simulink model "adc_16g_asnt"  (R2018a)
settings: Solver=VariableStepAuto  StartTime=0.0  StopTime=10.0  RelTol=1e-3
libraries: xbsIndex_r4 x65
settings Model: Creator=jkocz  LastModifiedBy=wei
settings CodeAppCC: StateflowObjectComments=on

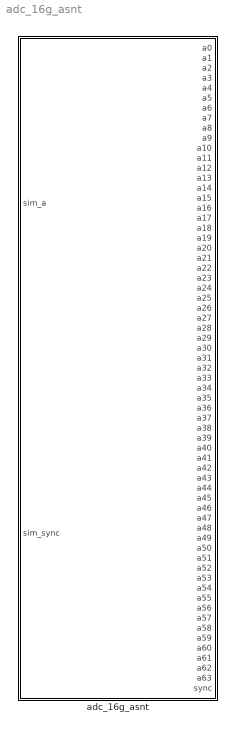
== system adc_16g_asnt ==
  adc_16g_asnt : Subsystem  Tag=xps:adc_4x16g_asnt  AncestorBlock=xps_adc/ADCs/adc_5g_e2v  mask(asnt_16g_adc){channel_sel=0}
      mask prompts: channel_sel "Channel Selection"
      mask init:
      | adc_16g_asnt_init(gcb);
      mask TypeOptions channel_sel: 0 | 1 | 2 | 3

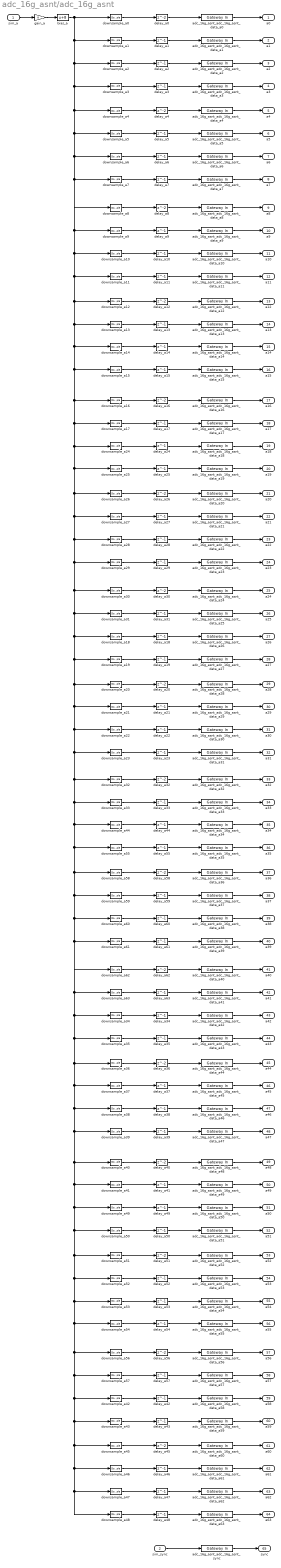
== system adc_16g_asnt/adc_16g_asnt ==
  sim_a : Inport
  sim_sync : Inport  Port=2
  adc_16g_asnt_adc_16g_asnt_data_a{0..63} (64 alike) : xbsIndex_r4/Gateway In  gui_display_data_type=Fixed-point  arith_type=Unsigned  n_bits=4  bin_pt=0  preci_type=Single  exp_width=8  frac_width=24  rows=1  columns=1  quantization=Truncate  overflow=Wrap  period=1  UseAsADC=off  ADCChannel='1'  interface=None  automatic_assignment=on  address_offset=hex2dec('00')  intf_name=''  intf_description=''  default_value=0  timing_constraint=None  locs_specified=off  LOCs={}  io_standard={}  inherit_from_input=off  hdl_port=on  dbl_ovrd=off  block_type=gatewayin
  adc_16g_asnt_adc_16g_asnt_sync : xbsIndex_r4/Gateway In  gui_display_data_type=Fixed-point  arith_type=Boolean  n_bits=16  bin_pt=14  preci_type=Single  exp_width=8  frac_width=24  rows=1  columns=1  quantization="Round  (unbiased: +/- Inf)"  overflow=Saturate  period=1  UseAsADC=off  ADCChannel='1'  interface=None  automatic_assignment=on  address_offset=hex2dec('00')  intf_name=''  intf_description=''  default_value=0  timing_constraint=None  locs_specified=off  LOCs={}  io_standard={}  inherit_from_input=off  hdl_port=on  dbl_ovrd=off  block_type=gatewayin
  bias_a : Bias  Bias=8  SaturateOnIntegerOverflow=on
  delay_a{0,4,8,12,16,20,26,30,32,36,40,45,51,56,58,62} (16 alike) : Delay  InitialCondition=0  InputProcessing=Inherited
  delay_a{1..3,5..7,9..11,13..15,17..19,21..25,27..29,31,33..35,37..39,41..44,46..50,52..55,57,59..61,63} (48 alike) : Delay  DelayLength=1  InitialCondition=0  InputProcessing=Inherited
  downsample_a{0,4,8,12,16,20,26,30,32,36,40,45,51,56,58,62} (16 alike) : DownSample  N=64  RateOptions=Allow multirate processing
  downsample_a{1,5,9,13,17,21,27,31,33,37,41,46,52,57,59,63} (16 alike) : DownSample  N=64  phase=1  RateOptions=Allow multirate processing
  downsample_a{2,6,10,14,18,22,24,28,34,38,42,44,47,49,53,60} (16 alike) : DownSample  N=64  phase=2  RateOptions=Allow multirate processing
  downsample_a{3,7,11,15,19,23,25,29,35,39,43,48,50,54..55,61} (16 alike) : DownSample  N=64  phase=3  RateOptions=Allow multirate processing
  gain_a : Gain  Gain=8  SaturateOnIntegerOverflow=on  OutDataTypeStr=Inherit: Same as input  ParamDataTypeStr=Inherit: Same as input
  a0 : Outport
  a1 : Outport  Port=2
  a2 : Outport  Port=3
  a3 : Outport  Port=4
  a4 : Outport  Port=5
  a5 : Outport  Port=6
  a6 : Outport  Port=7
  a7 : Outport  Port=8
  a8 : Outport  Port=9
  a9 : Outport  Port=10
  a10 : Outport  Port=11
  a11 : Outport  Port=12
  a12 : Outport  Port=13
  a13 : Outport  Port=14
  a14 : Outport  Port=15
  a15 : Outport  Port=16
  a16 : Outport  Port=17
  a17 : Outport  Port=18
  a18 : Outport  Port=19
  a19 : Outport  Port=20
  a20 : Outport  Port=21
  a21 : Outport  Port=22
  a22 : Outport  Port=23
  a23 : Outport  Port=24
  a24 : Outport  Port=25
  a25 : Outport  Port=26
  a26 : Outport  Port=27
  a27 : Outport  Port=28
  a28 : Outport  Port=29
  a29 : Outport  Port=30
  a30 : Outport  Port=31
  a31 : Outport  Port=32
  a32 : Outport  Port=33
  a33 : Outport  Port=34
  a34 : Outport  Port=35
  a35 : Outport  Port=36
  a36 : Outport  Port=37
  a37 : Outport  Port=38
  a38 : Outport  Port=39
  a39 : Outport  Port=40
  a40 : Outport  Port=41
  a41 : Outport  Port=42
  a42 : Outport  Port=43
  a43 : Outport  Port=44
  a44 : Outport  Port=45
  a45 : Outport  Port=46
  a46 : Outport  Port=47
  a47 : Outport  Port=48
  a48 : Outport  Port=49
  a49 : Outport  Port=50
  a50 : Outport  Port=51
  a51 : Outport  Port=52
  a52 : Outport  Port=53
  a53 : Outport  Port=54
  a54 : Outport  Port=55
  a55 : Outport  Port=56
  a56 : Outport  Port=57
  a57 : Outport  Port=58
  a58 : Outport  Port=59
  a59 : Outport  Port=60
  a60 : Outport  Port=61
  a61 : Outport  Port=62
  a62 : Outport  Port=63
  a63 : Outport  Port=64
  sync : Outport  Port=65
  wires:
  sim_sync/1 -> adc_16g_asnt_adc_16g_asnt_sync/1
  adc_16g_asnt_adc_16g_asnt_data_a3/1 -> a3/1
  delay_a3/1 -> adc_16g_asnt_adc_16g_asnt_data_a3/1
  downsample_a3/1 -> delay_a3/1
  adc_16g_asnt_adc_16g_asnt_data_a2/1 -> a2/1
  delay_a2/1 -> adc_16g_asnt_adc_16g_asnt_data_a2/1
  downsample_a2/1 -> delay_a2/1
  adc_16g_asnt_adc_16g_asnt_data_a1/1 -> a1/1
  delay_a1/1 -> adc_16g_asnt_adc_16g_asnt_data_a1/1
  downsample_a1/1 -> delay_a1/1
  adc_16g_asnt_adc_16g_asnt_data_a0/1 -> a0/1
  delay_a0/1 -> adc_16g_asnt_adc_16g_asnt_data_a0/1
  downsample_a0/1 -> delay_a0/1
  gain_a/1 -> bias_a/1
  sim_a/1 -> gain_a/1
  adc_16g_asnt_adc_16g_asnt_data_a6/1 -> a6/1
  delay_a4/1 -> adc_16g_asnt_adc_16g_asnt_data_a4/1
  adc_16g_asnt_adc_16g_asnt_data_a7/1 -> a7/1
  downsample_a5/1 -> delay_a5/1
  adc_16g_asnt_adc_16g_asnt_data_a4/1 -> a4/1
  downsample_a7/1 -> delay_a7/1
  adc_16g_asnt_adc_16g_asnt_data_a5/1 -> a5/1
  downsample_a6/1 -> delay_a6/1
  delay_a5/1 -> adc_16g_asnt_adc_16g_asnt_data_a5/1
  delay_a7/1 -> adc_16g_asnt_adc_16g_asnt_data_a7/1
  delay_a6/1 -> adc_16g_asnt_adc_16g_asnt_data_a6/1
  downsample_a4/1 -> delay_a4/1
  adc_16g_asnt_adc_16g_asnt_data_a10/1 -> a10/1
  delay_a8/1 -> adc_16g_asnt_adc_16g_asnt_data_a8/1
  adc_16g_asnt_adc_16g_asnt_data_a11/1 -> a11/1
  downsample_a9/1 -> delay_a9/1
  adc_16g_asnt_adc_16g_asnt_data_a8/1 -> a8/1
  downsample_a11/1 -> delay_a11/1
  adc_16g_asnt_adc_16g_asnt_data_a9/1 -> a9/1
  downsample_a10/1 -> delay_a10/1
  delay_a9/1 -> adc_16g_asnt_adc_16g_asnt_data_a9/1
  delay_a11/1 -> adc_16g_asnt_adc_16g_asnt_data_a11/1
  delay_a10/1 -> adc_16g_asnt_adc_16g_asnt_data_a10/1
  downsample_a8/1 -> delay_a8/1
  adc_16g_asnt_adc_16g_asnt_data_a14/1 -> a14/1
  delay_a12/1 -> adc_16g_asnt_adc_16g_asnt_data_a12/1
  adc_16g_asnt_adc_16g_asnt_data_a15/1 -> a15/1
  downsample_a13/1 -> delay_a13/1
  adc_16g_asnt_adc_16g_asnt_data_a12/1 -> a12/1
  downsample_a15/1 -> delay_a15/1
  adc_16g_asnt_adc_16g_asnt_data_a13/1 -> a13/1
  downsample_a14/1 -> delay_a14/1
  delay_a13/1 -> adc_16g_asnt_adc_16g_asnt_data_a13/1
  delay_a15/1 -> adc_16g_asnt_adc_16g_asnt_data_a15/1
  delay_a14/1 -> adc_16g_asnt_adc_16g_asnt_data_a14/1
  downsample_a12/1 -> delay_a12/1
  delay_a25/1 -> adc_16g_asnt_adc_16g_asnt_data_a19/1
  delay_a31/1 -> adc_16g_asnt_adc_16g_asnt_data_a25/1
  adc_16g_asnt_adc_16g_asnt_data_a27/1 -> a27/1
  adc_16g_asnt_adc_16g_asnt_data_a21/1 -> a21/1
  downsample_a29/1 -> delay_a29/1
  downsample_a27/1 -> delay_a27/1
  adc_16g_asnt_adc_16g_asnt_data_a20/1 -> a20/1
  adc_16g_asnt_adc_16g_asnt_data_a31/1 -> a31/1
  delay_a18/1 -> adc_16g_asnt_adc_16g_asnt_data_a26/1
  downsample_a21/1 -> delay_a21/1
  adc_16g_asnt_adc_16g_asnt_data_a25/1 -> a25/1
  adc_16g_asnt_adc_16g_asnt_data_a22/1 -> a22/1
  adc_16g_asnt_adc_16g_asnt_data_a18/1 -> a18/1
  downsample_a19/1 -> delay_a19/1
  delay_a23/1 -> adc_16g_asnt_adc_16g_asnt_data_a31/1
  downsample_a22/1 -> delay_a22/1
  downsample_a26/1 -> delay_a26/1
  delay_a28/1 -> adc_16g_asnt_adc_16g_asnt_data_a22/1
  delay_a21/1 -> adc_16g_asnt_adc_16g_asnt_data_a29/1
  delay_a30/1 -> adc_16g_asnt_adc_16g_asnt_data_a24/1
  downsample_a18/1 -> delay_a18/1
  downsample_a30/1 -> delay_a30/1
  downsample_a28/1 -> delay_a28/1
  downsample_a31/1 -> delay_a31/1
  delay_a27/1 -> adc_16g_asnt_adc_16g_asnt_data_a21/1
  delay_a22/1 -> adc_16g_asnt_adc_16g_asnt_data_a30/1
  adc_16g_asnt_adc_16g_asnt_data_a24/1 -> a24/1
  delay_a20/1 -> adc_16g_asnt_adc_16g_asnt_data_a28/1
  downsample_a20/1 -> delay_a20/1
  downsample_a23/1 -> delay_a23/1
  adc_16g_asnt_adc_16g_asnt_data_a26/1 -> a26/1
  adc_16g_asnt_adc_16g_asnt_data_a29/1 -> a29/1
  delay_a19/1 -> adc_16g_asnt_adc_16g_asnt_data_a27/1
  delay_a29/1 -> adc_16g_asnt_adc_16g_asnt_data_a23/1
  adc_16g_asnt_adc_16g_asnt_data_a23/1 -> a23/1
  downsample_a25/1 -> delay_a25/1
  downsample_a24/1 -> delay_a24/1
  adc_16g_asnt_adc_16g_asnt_data_a17/1 -> a17/1
  delay_a17/1 -> adc_16g_asnt_adc_16g_asnt_data_a17/1
  adc_16g_asnt_adc_16g_asnt_data_a16/1 -> a16/1
  downsample_a17/1 -> delay_a17/1
  adc_16g_asnt_adc_16g_asnt_data_a19/1 -> a19/1
  delay_a16/1 -> adc_16g_asnt_adc_16g_asnt_data_a16/1
  delay_a24/1 -> adc_16g_asnt_adc_16g_asnt_data_a18/1
  downsample_a16/1 -> delay_a16/1
  adc_16g_asnt_adc_16g_asnt_data_a28/1 -> a28/1
  adc_16g_asnt_adc_16g_asnt_data_a30/1 -> a30/1
  delay_a26/1 -> adc_16g_asnt_adc_16g_asnt_data_a20/1
  downsample_a59/1 -> delay_a59/1
  delay_a42/1 -> adc_16g_asnt_adc_16g_asnt_data_a58/1
  adc_16g_asnt_adc_16g_asnt_data_a36/1 -> a36/1
  adc_16g_asnt_adc_16g_asnt_data_a38/1 -> a38/1
  adc_16g_asnt_adc_16g_asnt_data_a42/1 -> a42/1
  downsample_a61/1 -> delay_a61/1
  downsample_a46/1 -> delay_a46/1
  delay_a53/1 -> adc_16g_asnt_adc_16g_asnt_data_a54/1
  downsample_a37/1 -> delay_a37/1
  delay_a39/1 -> adc_16g_asnt_adc_16g_asnt_data_a47/1
  downsample_a49/1 -> delay_a49/1
  adc_16g_asnt_adc_16g_asnt_data_a56/1 -> a56/1
  downsample_a50/1 -> delay_a50/1
  delay_a37/1 -> adc_16g_asnt_adc_16g_asnt_data_a45/1
  adc_16g_asnt_adc_16g_asnt_data_a47/1 -> a47/1
  delay_a34/1 -> adc_16g_asnt_adc_16g_asnt_data_a42/1
  downsample_a63/1 -> delay_a63/1
  delay_a50/1 -> adc_16g_asnt_adc_16g_asnt_data_a51/1
  downsample_a43/1 -> delay_a43/1
  downsample_a42/1 -> delay_a42/1
  delay_a38/1 -> adc_16g_asnt_adc_16g_asnt_data_a46/1
  downsample_a45/1 -> delay_a45/1
  downsample_a52/1 -> delay_a52/1
  downsample_a58/1 -> delay_a58/1
  downsample_a35/1 -> delay_a35/1
  adc_16g_asnt_adc_16g_asnt_data_a62/1 -> a62/1
  downsample_a56/1 -> delay_a56/1
  downsample_a54/1 -> delay_a54/1
  delay_a62/1 -> adc_16g_asnt_adc_16g_asnt_data_a40/1
  delay_a61/1 -> adc_16g_asnt_adc_16g_asnt_data_a39/1
  adc_16g_asnt_adc_16g_asnt_data_a60/1 -> a60/1
  adc_16g_asnt_adc_16g_asnt_data_a37/1 -> a37/1
  delay_a56/1 -> adc_16g_asnt_adc_16g_asnt_data_a56/1
  downsample_a60/1 -> delay_a60/1
  delay_a63/1 -> adc_16g_asnt_adc_16g_asnt_data_a41/1
  delay_a47/1 -> adc_16g_asnt_adc_16g_asnt_data_a62/1
  adc_16g_asnt_adc_16g_asnt_data_a43/1 -> a43/1
  downsample_a51/1 -> delay_a51/1
  downsample_a40/1 -> delay_a40/1
  adc_16g_asnt_adc_16g_asnt_data_a40/1 -> a40/1
  adc_16g_asnt_adc_16g_asnt_data_a61/1 -> a61/1
  adc_16g_asnt_adc_16g_asnt_data_a53/1 -> a53/1
  adc_16g_asnt_adc_16g_asnt_data_a63/1 -> a63/1
  adc_16g_asnt_adc_16g_asnt_data_a55/1 -> a55/1
  downsample_a62/1 -> delay_a62/1
  delay_a41/1 -> adc_16g_asnt_adc_16g_asnt_data_a49/1
  adc_16g_asnt_adc_16g_asnt_data_a39/1 -> a39/1
  adc_16g_asnt_adc_16g_asnt_data_a52/1 -> a52/1
  delay_a60/1 -> adc_16g_asnt_adc_16g_asnt_data_a38/1
  delay_a46/1 -> adc_16g_asnt_adc_16g_asnt_data_a61/1
  delay_a59/1 -> adc_16g_asnt_adc_16g_asnt_data_a37/1
  adc_16g_asnt_adc_16g_asnt_data_a58/1 -> a58/1
  adc_16g_asnt_adc_16g_asnt_data_a48/1 -> a48/1
  delay_a45/1 -> adc_16g_asnt_adc_16g_asnt_data_a60/1
  delay_a35/1 -> adc_16g_asnt_adc_16g_asnt_data_a43/1
  delay_a36/1 -> adc_16g_asnt_adc_16g_asnt_data_a44/1
  adc_16g_asnt_adc_16g_asnt_data_a57/1 -> a57/1
  downsample_a39/1 -> delay_a39/1
  downsample_a32/1 -> delay_a32/1
  downsample_a34/1 -> delay_a34/1
  downsample_a38/1 -> delay_a38/1
  adc_16g_asnt_adc_16g_asnt_data_a44/1 -> a44/1
  downsample_a36/1 -> delay_a36/1
  adc_16g_asnt_adc_16g_asnt_data_a59/1 -> a59/1
  delay_a40/1 -> adc_16g_asnt_adc_16g_asnt_data_a48/1
  delay_a48/1 -> adc_16g_asnt_adc_16g_asnt_data_a63/1
  adc_16g_asnt_adc_16g_asnt_data_a41/1 -> a41/1
  adc_16g_asnt_adc_16g_asnt_data_a45/1 -> a45/1
  downsample_a41/1 -> delay_a41/1
  adc_16g_asnt_adc_16g_asnt_data_a50/1 -> a50/1
  downsample_a47/1 -> delay_a47/1
  delay_a32/1 -> adc_16g_asnt_adc_16g_asnt_data_a32/1
  adc_16g_asnt_adc_16g_asnt_data_a51/1 -> a51/1
  adc_16g_asnt_adc_16g_asnt_data_a49/1 -> a49/1
  downsample_a53/1 -> delay_a53/1
  delay_a52/1 -> adc_16g_asnt_adc_16g_asnt_data_a53/1
  downsample_a57/1 -> delay_a57/1
  adc_16g_asnt_adc_16g_asnt_data_a54/1 -> a54/1
  delay_a43/1 -> adc_16g_asnt_adc_16g_asnt_data_a59/1
  delay_a49/1 -> adc_16g_asnt_adc_16g_asnt_data_a50/1
  delay_a57/1 -> adc_16g_asnt_adc_16g_asnt_data_a57/1
  delay_a51/1 -> adc_16g_asnt_adc_16g_asnt_data_a52/1
  downsample_a55/1 -> delay_a55/1
  downsample_a44/1 -> delay_a44/1
  adc_16g_asnt_adc_16g_asnt_data_a33/1 -> a33/1
  delay_a33/1 -> adc_16g_asnt_adc_16g_asnt_data_a33/1
  adc_16g_asnt_adc_16g_asnt_data_a32/1 -> a32/1
  downsample_a33/1 -> delay_a33/1
  adc_16g_asnt_adc_16g_asnt_data_a35/1 -> a35/1
  bias_a/1 -> downsample_a44/1, downsample_a46/1, downsample_a47/1, downsample_a48/1, downsample_a45/1, downsample_a43/1, downsample_a42/1, downsample_a57/1, downsample_a56/1, downsample_a54/1, downsample_a53/1, downsample_a52/1, downsample_a51/1, downsample_a50/1, downsample_a49/1, downsample_a41/1, downsample_a40/1, downsample_a39/1, downsample_a38/1, downsample_a37/1, downsample_a36/1, downsample_a35/1, downsample_a34/1, downsample_a63/1, downsample_a32/1, downsample_a33/1, downsample_a55/1, downsample_a58/1, downsample_a59/1, downsample_a60/1, downsample_a62/1, downsample_a61/1, downsample_a23/1, downsample_a22/1, downsample_a21/1, downsample_a20/1, downsample_a19/1, downsample_a18/1, downsample_a31/1, downsample_a30/1, downsample_a29/1, downsample_a28/1, downsample_a27/1, downsample_a26/1, downsample_a25/1, downsample_a24/1, downsample_a17/1, downsample_a16/1, downsample_a15/1, downsample_a14/1, downsample_a13/1, downsample_a12/1, downsample_a11/1, downsample_a10/1, downsample_a9/1, downsample_a2/1, downsample_a0/1, downsample_a1/1, downsample_a3/1, downsample_a4/1, downsample_a5/1, downsample_a6/1, downsample_a8/1, downsample_a7/1
  downsample_a48/1 -> delay_a48/1
  delay_a55/1 -> adc_16g_asnt_adc_16g_asnt_data_a35/1
  adc_16g_asnt_adc_16g_asnt_data_a34/1 -> a34/1
  delay_a44/1 -> adc_16g_asnt_adc_16g_asnt_data_a34/1
  delay_a54/1 -> adc_16g_asnt_adc_16g_asnt_data_a55/1
  adc_16g_asnt_adc_16g_asnt_data_a46/1 -> a46/1
  delay_a58/1 -> adc_16g_asnt_adc_16g_asnt_data_a36/1
  adc_16g_asnt_adc_16g_asnt_sync/1 -> sync/1
